simulink model "beacon_approach"  (R2025b)
settings: Solver=VariableStepAuto  StartTime=0.0  StopTime=Stop_Time  MaxStep=1e-3  RelTol=1e-3
values from neighbouring files (symbols this model uses):
  CAM_LATENCY_S = 0.35    [robot_params.m]
  K_phi = 0.471    [robot_params.m]
  K_rho = 0.0825    [robot_params.m]
  Ki_phi = 2.0    (= 2)    [robot_params.m]
  Ki_rho = 2.0    (= 2)    [robot_params.m]
  Kp_phi = 4.0    (= 4)    [robot_params.m]
  Kp_phi_dot = 8.5    [robot_params.m]
  Kp_rho = 3.0    (= 3)    [robot_params.m]
  Kp_rho_dot = 48.0    (= 48)    [robot_params.m]
  MAX_VOLTAGE = 6.0    (= 6)    [robot_params.m]
  PHI_DOT_LIMIT = 6.75    [robot_params.m]
  RHO_DOT_LIMIT = 1.125    [robot_params.m]
  sigma_phi = 5    [robot_params.m]
  sigma_rho = 5    [robot_params.m]
  Ts = 0.01    [robot_params.m]
libraries: simulink x1
settings Model: Creator=henry  LastModifiedBy=henry

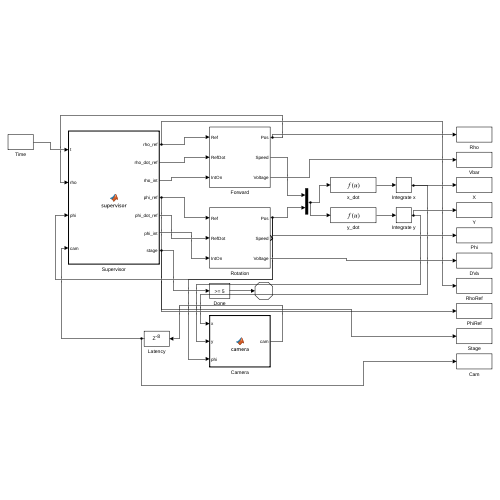
[thumbnail: Simulink's stored preview of the top-level diagram]
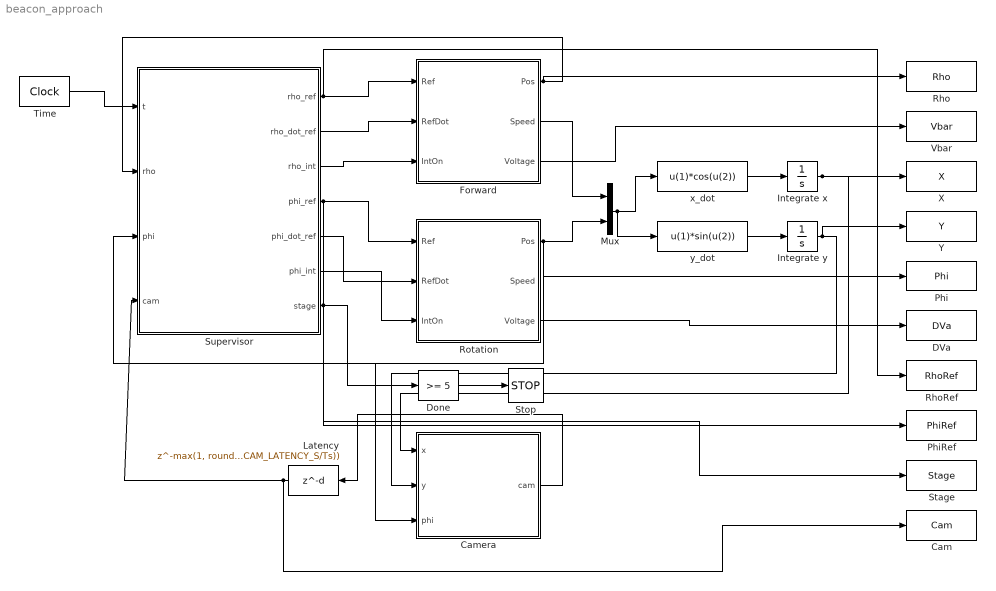
== system beacon_approach ==
  Cam : ToWorkspace  VariableName=Cam  SaveFormat=Timeseries  SampleTime=-1
  Camera : MATLAB Function  TreatAsAtomicUnit=on
  DVa : ToWorkspace  VariableName=DVa  SaveFormat=Timeseries  SampleTime=-1
  Done : simulink/Logic and Bit Operations/Compare To Constant  relop=>=  const=5  OutDataTypeStr=boolean
  Forward : Subsystem
  Integrate x : Integrator
  Integrate y : Integrator
  Latency : Delay  DelayLength=max(1, round(CAM_LATENCY_S/Ts))  InitialCondition=0  SampleTime=Ts
  Mux : Mux  Inputs=2
  Phi : ToWorkspace  VariableName=Phi  SaveFormat=Timeseries  SampleTime=-1
  PhiRef : ToWorkspace  VariableName=PhiRef  SaveFormat=Timeseries  SampleTime=-1
  Rho : ToWorkspace  VariableName=Rho  SaveFormat=Timeseries  SampleTime=-1
  RhoRef : ToWorkspace  VariableName=RhoRef  SaveFormat=Timeseries  SampleTime=-1
  Rotation : Subsystem
  Stage : ToWorkspace  VariableName=Stage  SaveFormat=Timeseries  SampleTime=-1
  Stop : Stop
  Supervisor : MATLAB Function  TreatAsAtomicUnit=on
  Time : DigitalClock  SampleTime=Ts
  Vbar : ToWorkspace  VariableName=Vbar  SaveFormat=Timeseries  SampleTime=-1
  X : ToWorkspace  VariableName=X  SaveFormat=Timeseries  SampleTime=-1
  Y : ToWorkspace  VariableName=Y  SaveFormat=Timeseries  SampleTime=-1
  x_dot : Fcn  Expr=u(1)*cos(u(2))
  y_dot : Fcn  Expr=u(1)*sin(u(2))
  wires:
  Time/1 -> Supervisor/1(t)
  Supervisor/1(rho_ref) -> Forward/1(Ref), RhoRef/1
  Supervisor/4(phi_ref) -> Rotation/1(Ref), PhiRef/1
  Supervisor/2(rho_dot_ref) -> Forward/2(RefDot)
  Supervisor/5(phi_dot_ref) -> Rotation/2(RefDot)
  Supervisor/3(rho_int) -> Forward/3(IntOn)
  Supervisor/6(phi_int) -> Rotation/3(IntOn)
  Forward/2(Speed) -> Mux/1
  Rotation/1(Pos) -> Mux/2, Camera/3(phi), Supervisor/3(phi), Phi/1
  Mux/1 -> x_dot/1, y_dot/1
  x_dot/1 -> Integrate x/1
  y_dot/1 -> Integrate y/1
  Integrate x/1 -> Camera/1(x), X/1
  Integrate y/1 -> Camera/2(y), Y/1
  Camera/1(cam) -> Latency/1
  Latency/1 -> Supervisor/4(cam), Cam/1
  Forward/1(Pos) -> Supervisor/2(rho), Rho/1
  Supervisor/7(stage) -> Done/1, Stage/1
  Done/1 -> Stop/1
  Forward/3(Voltage) -> Vbar/1
  Rotation/3(Voltage) -> DVa/1

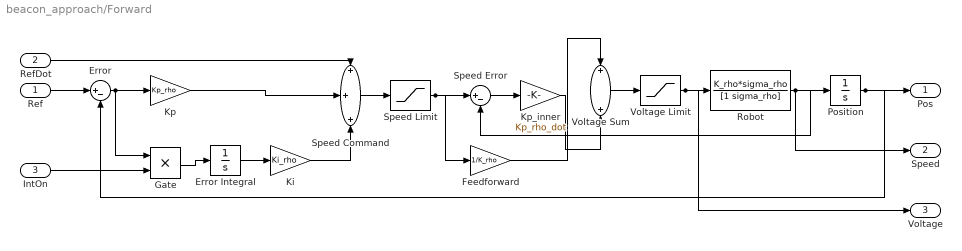
== system beacon_approach/Forward ==
  Ref : Inport
  RefDot : Inport  Port=2
  IntOn : Inport  Port=3
  Error : Sum  Inputs=|+-
  Error Integral : Integrator
  Feedforward : Gain  Gain=1/K_rho
  Gate : Product
  Ki : Gain  Gain=Ki_rho
  Kp : Gain  Gain=Kp_rho
  Kp_inner : Gain  Gain=Kp_rho_dot
  Position : Integrator
  Robot : TransferFcn  Numerator=K_rho*sigma_rho  Denominator=[1 sigma_rho]
  Speed Command : Sum  Inputs=+++
  Speed Error : Sum  Inputs=|+-
  Speed Limit : Saturate  UpperLimit=RHO_DOT_LIMIT  LowerLimit=-RHO_DOT_LIMIT
  Voltage Limit : Saturate  UpperLimit=2*MAX_VOLTAGE  LowerLimit=-2*MAX_VOLTAGE
  Voltage Sum : Sum
  Pos : Outport
  Speed : Outport  Port=2
  Voltage : Outport  Port=3
  wires:
  Ref/1 -> Error/1
  Position/1 -> Error/2, Pos/1
  Error/1 -> Kp/1, Gate/1
  IntOn/1 -> Gate/2
  Gate/1 -> Error Integral/1
  Error Integral/1 -> Ki/1
  RefDot/1 -> Speed Command/1
  Kp/1 -> Speed Command/2
  Ki/1 -> Speed Command/3
  Speed Command/1 -> Speed Limit/1
  Speed Limit/1 -> Feedforward/1, Speed Error/1
  Robot/1 -> Speed Error/2, Position/1, Speed/1
  Speed Error/1 -> Kp_inner/1
  Feedforward/1 -> Voltage Sum/1
  Kp_inner/1 -> Voltage Sum/2
  Voltage Sum/1 -> Voltage Limit/1
  Voltage Limit/1 -> Robot/1, Voltage/1

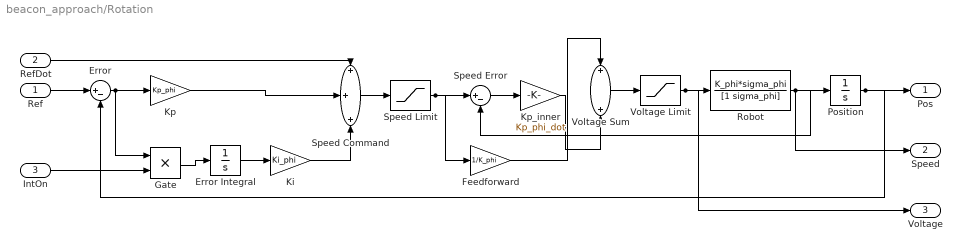
== system beacon_approach/Rotation ==
  Ref : Inport
  RefDot : Inport  Port=2
  IntOn : Inport  Port=3
  Error : Sum  Inputs=|+-
  Error Integral : Integrator
  Feedforward : Gain  Gain=1/K_phi
  Gate : Product
  Ki : Gain  Gain=Ki_phi
  Kp : Gain  Gain=Kp_phi
  Kp_inner : Gain  Gain=Kp_phi_dot
  Position : Integrator
  Robot : TransferFcn  Numerator=K_phi*sigma_phi  Denominator=[1 sigma_phi]
  Speed Command : Sum  Inputs=+++
  Speed Error : Sum  Inputs=|+-
  Speed Limit : Saturate  UpperLimit=PHI_DOT_LIMIT  LowerLimit=-PHI_DOT_LIMIT
  Voltage Limit : Saturate  UpperLimit=2*MAX_VOLTAGE  LowerLimit=-2*MAX_VOLTAGE
  Voltage Sum : Sum
  Pos : Outport
  Speed : Outport  Port=2
  Voltage : Outport  Port=3
  wires:
  Ref/1 -> Error/1
  Position/1 -> Error/2, Pos/1
  Error/1 -> Kp/1, Gate/1
  IntOn/1 -> Gate/2
  Gate/1 -> Error Integral/1
  Error Integral/1 -> Ki/1
  RefDot/1 -> Speed Command/1
  Kp/1 -> Speed Command/2
  Ki/1 -> Speed Command/3
  Speed Command/1 -> Speed Limit/1
  Speed Limit/1 -> Feedforward/1, Speed Error/1
  Robot/1 -> Speed Error/2, Position/1, Speed/1
  Speed Error/1 -> Kp_inner/1
  Feedforward/1 -> Voltage Sum/1
  Kp_inner/1 -> Voltage Sum/2
  Voltage Sum/1 -> Voltage Limit/1
  Voltage Limit/1 -> Robot/1, Voltage/1

== matlab function beacon_approach/Camera ==
  settings: updateMethod=DISCRETE  sampleTime=Ts
  data: x input; cam output; y input; phi input; P parameter
function cam = camera(x, y, phi, P)
% The camera and Pi. See beacon_camera.m.
cam = beacon_camera(x, y, phi, P);

== matlab function beacon_approach/Supervisor ==
  settings: updateMethod=DISCRETE  sampleTime=Ts
  data: t input; rho_ref output; rho input; phi input; cam input; rho_dot_ref output; rho_int output; phi_ref output; phi_dot_ref output; phi_int output; stage output; P parameter
function [rho_ref, rho_dot_ref, rho_int, phi_ref, phi_dot_ref, phi_int, stage] = supervisor(t, rho, phi, cam, P)
% The stage logic of beacon.ino. See beacon_supervisor.m.
[rho_ref, rho_dot_ref, rho_int, phi_ref, phi_dot_ref, phi_int, stage] = beacon_supervisor(t, rho, phi, cam, P);
